simulink subsystem "quatNormalize"  (R2024b)
settings: Solver=VariableStepAuto  StartTime=0.0  StopTime=10.0  RelTol=1e-3
settings Model: Creator=pierb  LastModifiedBy=pierb

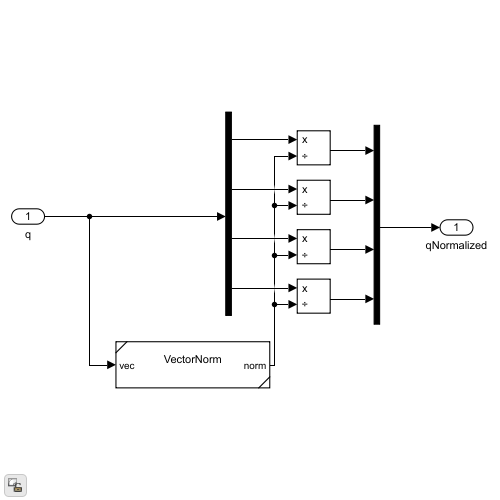
[thumbnail: Simulink's stored preview of the top-level diagram]
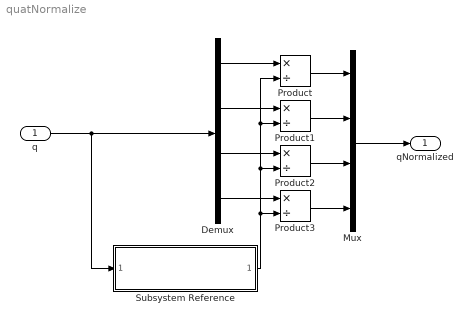
== system quatNormalize ==
  q : Inport
  Demux : Demux
  Mux : Mux
  Product{,1..3} (4 alike) : Product  Inputs=*/
  Subsystem Reference : Subsystem  ReferencedSubsystem=VectorNorm
  qNormalized : Outport  Unit=1  VectorParamsAs1DForOutWhenUnconnected=off
  wires:
  Product/1 -> Mux/1
  Subsystem Reference/1 -> Product3/2, Product2/2, Product/2, Product1/2
  q/1 -> Subsystem Reference/1, Demux/1
  Demux/3 -> Product2/1
  Demux/2 -> Product1/1
  Product2/1 -> Mux/3
  Mux/1 -> qNormalized/1
  Product1/1 -> Mux/2
  Product3/1 -> Mux/4
  Demux/1 -> Product/1
  Demux/4 -> Product3/1
